simulink model "mav_animation"  (R2025b)
settings: Solver=ode15s  StartTime=0.0  StopTime=10000  RelTol=1e-3  EnableMultiTasking=on
InitFcn:
  | pioneer_parameters
undefined symbols (not defined in the file or in its folder): AP, autopilot, drawAircraft, plotmavstatevariables, SIM, true_states, WIND
libraries: simulink x3
settings Model: Creator=beard  LastModifiedBy=rudra
settings SolverCC: AlgebraicLoopSolver=TrustRegion
settings DataIOCC: LimitDataPoints=on  SaveFormat=Array  SignalLoggingSaveFormat=ModelDataLogs  ReturnWorkspaceOutputs=off
settings OptimizationCC: ExpressionDepthLimit=2147483647.0  InitFltsAndDblsToZero=on  LifeSpan=inf
settings DebuggingCC: UnderspecifiedInitializationDetection=Classic  MergeDetectMultiDrivingBlocksExec=none  SolverPrmCheckMsg=warning  FcnCallInpInsideContextMsg=warning  UnconnectedInputMsg=warning  UnconnectedOutputMsg=warning  UnconnectedLineMsg=warning  AllowSymbolicDim=off  StateNameClashWarn=warning  SFUnexpectedBacktrackingDiag=warning  SFNoUnconditionalDefaultTransitionDiag=warning  SFExecutionAtInitializationDiag=none  ArithmeticOperatorsInVariantConditions=warning
settings HardwareCC: ProdBitPerPointer=32.0  ProdBitPerSizeT=32.0  ProdBitPerPtrDiffT=32.0  ProdLargestAtomicFloat=None  ProdIntDivRoundTo=Undefined  ProdEndianess=Unspecified  ProdWordSize=32.0  ProdHWDeviceType=32-bit Generic
settings ModelReferenceCC: EnableRefExpFcnMdlSchedulingChecks=on  PropagateSignalLabelsOutOfModel=off
settings SFSimCC: SimUseLocalCustomCode=off  CustomCodeUndefinedFunction=UseInterfaceOnly
settings RTWCC: RTWUseLocalCustomCode=off  GPUComputeCapability=3.5
settings CodeAppCC: StateflowObjectComments=on
settings GRTTargetCC: TargetLangStandard=C89/C90 (ANSI)  CombineOutputUpdateFcns=off  GRTInterface=on
settings ConfigComp: CovMetricSettings=dw  CovSaveCumulativeToWorkspaceVar=on  CovSaveSingleToWorkspaceVar=on  CovExternalEMLEnable=off  CovSFcnEnable=off

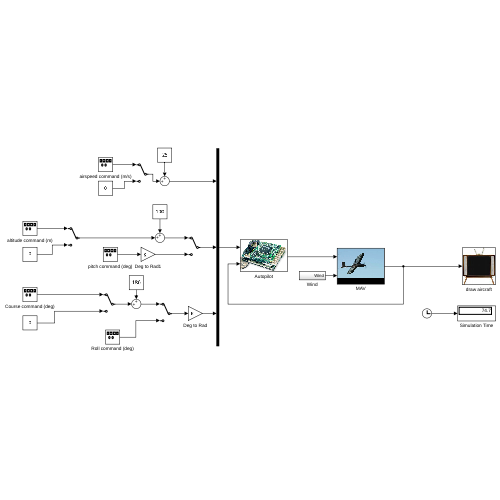
[thumbnail: Simulink's stored preview of the top-level diagram]
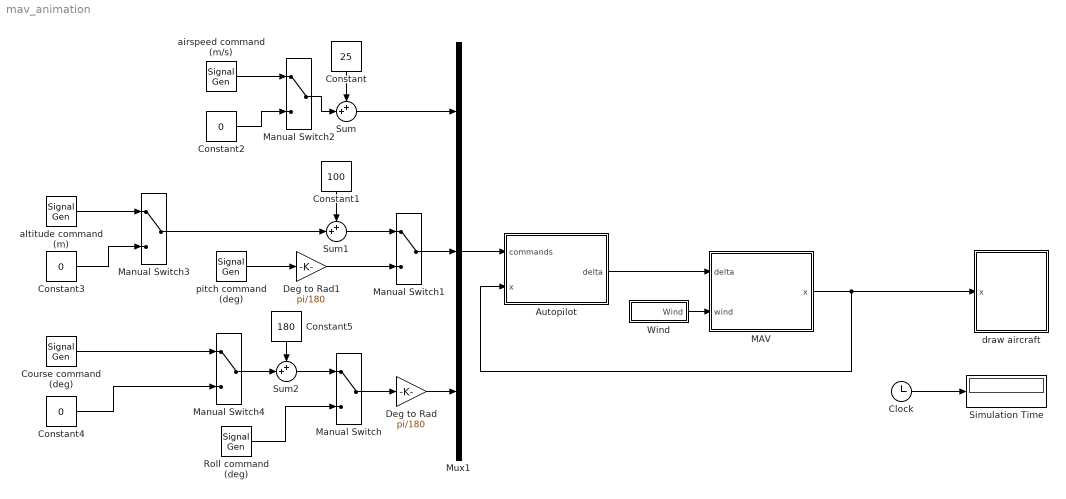
== system mav_animation ==
  Autopilot : Subsystem
      mask Display: image(imread('kestrel.jpg'))
  Clock : Clock
  Constant : Constant  Value=25
  Constant1 : Constant  Value=100
  Constant2 : Constant  Value=0
  Constant3 : Constant  Value=0
  Constant4 : Constant  Value=0
  Constant5 : Constant  Value=180
  Course command (deg) : SignalGenerator  WaveForm=square  Amplitude=45  Frequency=.02
  Deg to Rad : Gain  Gain=pi/180
  Deg to Rad1 : Gain  Gain=pi/180
  MAV : Subsystem
      mask Display: image(imread('batcam.png'))
  Manual Switch{,1..4} (5 alike) : ManualSwitch
  Mux1 : Mux  Inputs=3
  Roll command (deg) : SignalGenerator  WaveForm=square  Amplitude=20  Frequency=.1
  Simulation Time : Display
  Sum : Sum  Inputs=++|
  Sum1 : Sum  Inputs=++|
  Sum2 : Sum  Inputs=++|
  Wind : Subsystem
  airspeed command (m/s) : SignalGenerator  WaveForm=square  Amplitude=4  Frequency=.02
  altitude command (m) : SignalGenerator  WaveForm=square  Amplitude=10  Frequency=.02
  draw aircraft : Subsystem
      mask Display: image(imread('tv.jpg'))
  pitch command (deg) : SignalGenerator  WaveForm=square  Amplitude=10  Frequency=.05
  wires:
  Clock/1 -> Simulation Time/1
  Wind/1(Wind) -> MAV/2(wind)
  MAV/1(x) -> draw aircraft/1(x), Autopilot/2(x)
  Autopilot/1(delta) -> MAV/1(delta)
  Mux1/1 -> Autopilot/1(commands)
  Deg to Rad/1 -> Mux1/3
  pitch command (deg)/1 -> Deg to Rad1/1
  Roll command (deg)/1 -> Manual Switch/2
  Manual Switch1/1 -> Mux1/2
  Sum/1 -> Mux1/1
  Constant/1 -> Sum/1
  Sum1/1 -> Manual Switch1/1
  Constant1/1 -> Sum1/1
  Manual Switch/1 -> Deg to Rad/1
  Deg to Rad1/1 -> Manual Switch1/2
  Manual Switch2/1 -> Sum/2
  altitude command (m)/1 -> Manual Switch3/1
  airspeed command (m/s)/1 -> Manual Switch2/1
  Constant2/1 -> Manual Switch2/2
  Manual Switch3/1 -> Sum1/2
  Constant3/1 -> Manual Switch3/2
  Constant4/1 -> Manual Switch4/2
  Constant5/1 -> Sum2/1
  Sum2/1 -> Manual Switch/1
  Manual Switch4/1 -> Sum2/2
  Course command (deg)/1 -> Manual Switch4/1

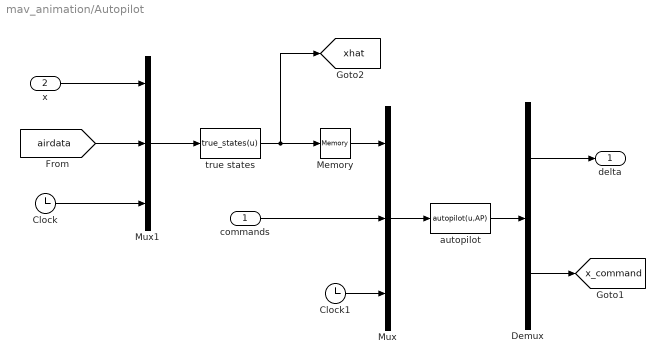
== system mav_animation/Autopilot ==
  commands : Inport
  x : Inport  Port=2
  Clock : Clock
  Clock1 : Clock
  Demux : Demux  Outputs=[4;12]
  Memory : Memory
  Mux : Mux  Inputs=3
  Mux1 : Mux  Inputs=3
  autopilot : MATLABFcn  MATLABFcn=autopilot(u,AP)  OutputDimensions=4+12  SampleTime=SIM.ts_simulation
  true states : MATLABFcn  MATLABFcn=true_states(u)  OutputDimensions=19  SampleTime=SIM.ts_simulation
  delta : Outport  VectorParamsAs1DForOutWhenUnconnected=off
  tag scope: x_command=global, xhat=global
  wires:
  Mux/1 -> autopilot/1
  Clock/1 -> Mux1/3
  autopilot/1 -> Demux/1
  Demux/1 -> delta/1
  Demux/2 -> [x_command]
  commands/1 -> Mux/2
  Mux1/1 -> true states/1
  x/1 -> Mux1/1
  true states/1 -> [xhat], Memory/1
  [airdata] -> Mux1/2
  Memory/1 -> Mux/1
  Clock1/1 -> Mux/3

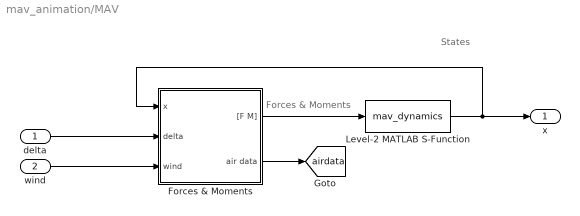
== system mav_animation/MAV ==
  note: Forces & Moments
  note: States
  delta : Inport
  wind : Inport  Port=2
  Forces & Moments : Subsystem
  Level-2 MATLAB S-Function : M-S-Function  FunctionName=mav_dynamics  Parameters=P
  x : Outport  VectorParamsAs1DForOutWhenUnconnected=off
  tag scope: airdata=global
  wires:
  Forces & Moments/1("[F M]") -> Level-2 MATLAB S-Function/1
  Forces & Moments/2(air data) -> [airdata]
  delta/1 -> Forces & Moments/2(delta)
  wind/1 -> Forces & Moments/3(wind)
  Level-2 MATLAB S-Function/1 -> Forces & Moments/1(x), x/1

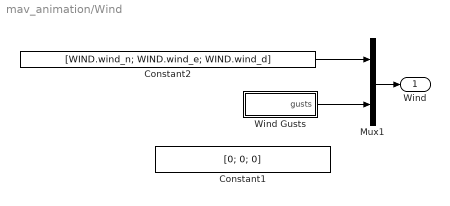
== system mav_animation/Wind ==
  Constant1 : Constant  Value=[0; 0; 0]
  Constant2 : Constant  Value=[WIND.wind_n; WIND.wind_e; WIND.wind_d]
  Mux1 : Mux  Inputs=2
  Wind Gusts : Subsystem
  Wind : Outport  VectorParamsAs1DForOutWhenUnconnected=off
  wires:
  Constant2/1 -> Mux1/1
  Mux1/1 -> Wind/1
  Wind Gusts/1(gusts) -> Mux1/2

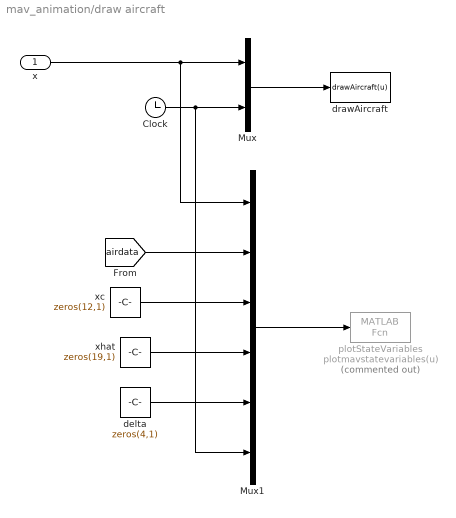
== system mav_animation/draw aircraft ==
  x : Inport
  Clock : Clock
  Mux : Mux  Inputs=2
  Mux1 : Mux  Inputs=6
  delta : Constant  Value=zeros(4,1)
  drawAircraft : MATLABFcn  MATLABFcn=drawAircraft(u)  OutputDimensions=0  SampleTime=0.1
  plotStateVariables : MATLABFcn  Commented=on  MATLABFcn=plotmavstatevariables(u)  OutputDimensions=0  SampleTime=0.1
  xc : Constant  Value=zeros(12,1)
  xhat : Constant  Value=zeros(19,1)
  wires:
  [airdata] -> Mux1/2
  delta/1 -> Mux1/5
  xc/1 -> Mux1/3
  xhat/1 -> Mux1/4
  Mux1/1 -> plotStateVariables/1
  Clock/1 -> Mux1/6, Mux/2
  x/1 -> Mux1/1, Mux/1
  Mux/1 -> drawAircraft/1

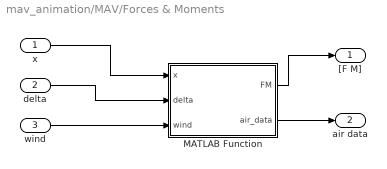
== system mav_animation/MAV/Forces & Moments ==
  x : Inport
  delta : Inport  Port=2
  wind : Inport  Port=3
  MATLAB Function : MATLAB Function  TreatAsAtomicUnit=on
  "[F M]" : Outport  VectorParamsAs1DForOutWhenUnconnected=off
  air data : Outport  Port=2  VectorParamsAs1DForOutWhenUnconnected=off
  wires:
  x/1 -> MATLAB Function/1(x)
  delta/1 -> MATLAB Function/2(delta)
  wind/1 -> MATLAB Function/3(wind)
  MATLAB Function/1(FM) -> "[F M]"/1
  MATLAB Function/2(air_data) -> air data/1

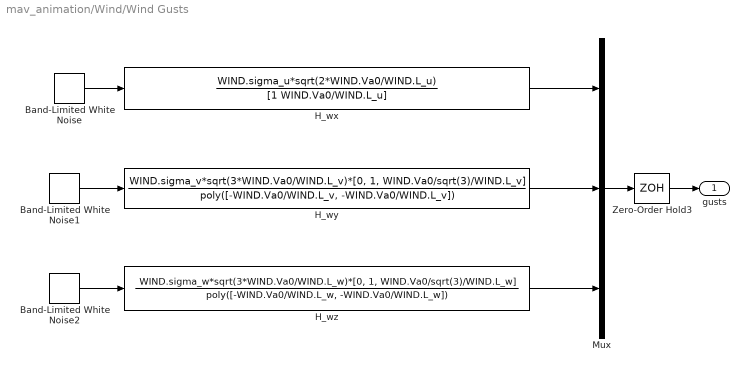
== system mav_animation/Wind/Wind Gusts ==
  Band-Limited White Noise : simulink/Sources/Band-Limited White Noise  Cov=[1]  Ts=SIM.ts_simulation  seed=[23341]
  Band-Limited White Noise1 : simulink/Sources/Band-Limited White Noise  Cov=[1]  Ts=SIM.ts_simulation  seed=[23341]
  Band-Limited White Noise2 : simulink/Sources/Band-Limited White Noise  Cov=[1]  Ts=SIM.ts_simulation  seed=[23341]
  H_wx : TransferFcn  Numerator=WIND.sigma_u*sqrt(2*WIND.Va0/WIND.L_u)  Denominator=[1 WIND.Va0/WIND.L_u]
  H_wy : TransferFcn  Numerator=WIND.sigma_v*sqrt(3*WIND.Va0/WIND.L_v)*[0, 1, WIND.Va0/sqrt(3)/WIND.L_v]  Denominator=poly([-WIND.Va0/WIND.L_v, -WIND.Va0/WIND.L_v])
  H_wz : TransferFcn  Numerator=WIND.sigma_w*sqrt(3*WIND.Va0/WIND.L_w)*[0, 1, WIND.Va0/sqrt(3)/WIND.L_w]  Denominator=poly([-WIND.Va0/WIND.L_w, -WIND.Va0/WIND.L_w])
  Mux : Mux  Inputs=3
  Zero-Order Hold3 : ZeroOrderHold  SampleTime=SIM.ts_simulation
  gusts : Outport  VectorParamsAs1DForOutWhenUnconnected=off
  wires:
  H_wx/1 -> Mux/1
  Band-Limited White Noise/1 -> H_wx/1
  H_wy/1 -> Mux/2
  Band-Limited White Noise1/1 -> H_wy/1
  H_wz/1 -> Mux/3
  Band-Limited White Noise2/1 -> H_wz/1
  Mux/1 -> Zero-Order Hold3/1
  Zero-Order Hold3/1 -> gusts/1

== matlab function mav_animation/MAV/Forces & Moments/MATLAB Function ==
  data: x input; FM output; delta input; wind input; air_data output; P parameter
function [FM, air_data] = fcn(x, delta, wind, P)
    % Pre-allocate outputs for the C-compiler
    FM = zeros(6,1);
    air_data = zeros(3,1);
    
    % Call your external file
    [FM, air_data] = forces_moments(x, delta, wind, P);
end
